simulink model "xz_packaging_automatic"  (R2025b)
settings: Solver=ode15s  StartTime=0.0  StopTime=10.45  MaxStep=0.001  RelTol=1e-6  AbsTol=1e-9
model workspace: external: MATLAB File xz_packaging_automatic_DataFile.m (data not in the file)
values from neighbouring files (symbols this model uses):
  payloadMass_kg = 0.25    [xz_packaging_automatic_DataFile.m]
undefined symbols (not defined in the file or in its folder): smiData, X, Y, Z
libraries: sm_lib x2549, nesl_utility x31
(part 1 of 38)
settings Model: Creator=Asus  LastModifiedBy=Asus

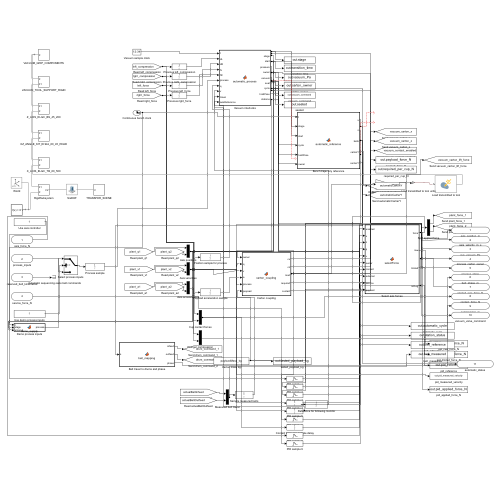
[thumbnail: Simulink's stored preview of the top-level diagram]
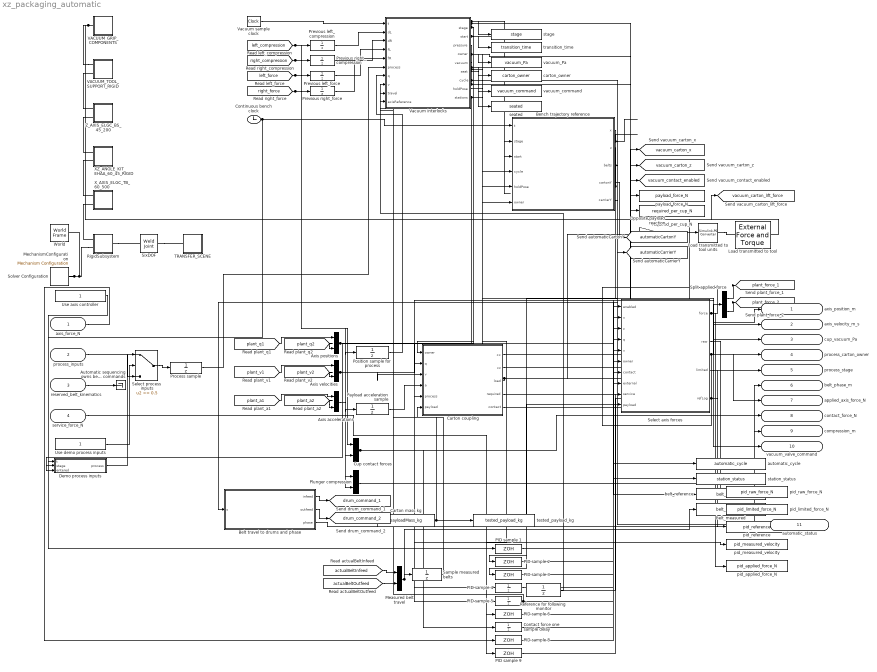
== system xz_packaging_automatic ==
  axis_force_N : Inport  PortDimensions=2
  process_inputs : Inport  Port=2  PortDimensions=12
  reserved_belt_kinematics : Inport  Port=3  PortDimensions=6
  service_force_N : Inport  Port=4  PortDimensions=2
  Automatic sequencing owns belt commands : Terminator
  Axis accelerations : Mux  Inputs=2
  Axis positions : Mux  Inputs=2
  Axis velocities : Mux  Inputs=2
  Belt travel to drums and phase : MATLAB Function  TreatAsAtomicUnit=on
  Bench trajectory reference : MATLAB Function  TreatAsAtomicUnit=on
  Carton coupling : MATLAB Function  TreatAsAtomicUnit=on
  Carton mass kg : Constant  Value=payloadMass_kg
  Contact force one sample delay : UnitDelay  SampleTime=0.001  HasFrameUpgradeWarning=on
  Continuous bench clock : Clock
  Cup contact forces : Mux  Inputs=2
  Demo process inputs : MATLAB Function  TreatAsAtomicUnit=on
  Load transmitted to tool : sm_lib/Forces and Torques/External Force and Torque  EnableForceX=off  EnableForceY=off  EnableForceZ=off  EnableForce=on  ForceResolutionFrame=World  EnableTorqueX=off  EnableTorqueY=off  EnableTorqueZ=off  EnableTorque=off  TorqueResolutionFrame=AttachedFrame
  Load transmitted to tool units : nesl_utility/Simulink-PS Converter  PhysicalDomain=network_engine_domain  SubClassName=ps_input  LeftPortType=input  RightPortType=output  PseudoPeriodic=off  Frequencies=[]  NoiseDistribution=none  NoiseParameters=[]  Unit=N  AffineConversion=off  FilteringAndDerivatives=provide  SimscapeFilterOrder=1  InputFilterTimeConstant=0.001  UdotUserProvided=0
  Measured belt travel : Mux  Inputs=2
  MechanismConfiguration : sm_lib/Utilities/Mechanism Configuration  UniformGravity=Constant  GravityVector=[0 0 -9.8066499999999994]  GravityVectorUnits=m/s^2  LinearizationDelta=0.001  JointModeTransitionNonlinearIterations=2
  Opposite payload reaction : Gain  Gain=-1
  PID sample {1..3,6,8..9} (6 alike) : ZeroOrderHold  SampleTime=0.001
  PID sample 4 : UnitDelay  InitialCondition=[0.05;0.024]  SampleTime=0.001  HasFrameUpgradeWarning=on
  PID sample 5 : UnitDelay  SampleTime=0.001  HasFrameUpgradeWarning=on
  Payload acceleration sample : UnitDelay  SampleTime=0.001  HasFrameUpgradeWarning=on
  Plunger compression : Mux  Inputs=2
  Position sample for process : UnitDelay  SampleTime=0.001  HasFrameUpgradeWarning=on
  Previous left_compression : UnitDelay  SampleTime=0.001  HasFrameUpgradeWarning=on
  Previous left_force : UnitDelay  SampleTime=0.001  HasFrameUpgradeWarning=on
  Previous right_compression : UnitDelay  SampleTime=0.001  HasFrameUpgradeWarning=on
  Previous right_force : UnitDelay  SampleTime=0.001  HasFrameUpgradeWarning=on
  Process sample : UnitDelay  SampleTime=0.001  HasFrameUpgradeWarning=on
  Reference for following monitor : UnitDelay  InitialCondition=[0.05 0 0;0.024 0 0]  SampleTime=0.001  HasFrameUpgradeWarning=on
  RigidSubsystem : Subsystem
  Sample measured belts : UnitDelay  SampleTime=0.001  HasFrameUpgradeWarning=on
  Select axis forces : MATLAB Function  TreatAsAtomicUnit=on
  Select process inputs : Switch  Threshold=0.5  SaturateOnIntegerOverflow=off  InputSameDT=off
  SixDOF : sm_lib/Joints/Weld Joint  JointMode=Normal  CompositeWrenchDir=FollowerOnBase  CompositeWrenchFrame=BaseFrame  SenseConstraintForce=off  SenseConstraintTorque=off  SenseTotalForce=off  SenseTotalTorque=off
  Solver Configuration : nesl_utility/Solver Configuration  PhysicalDomain=network_engine_domain  SubClassName=solver  LeftPortType=input  RightPortType=generic  Tones=[]  Harmonics=[]  SimulateNoise=off  Profile=off  UseLocalSampling=off  EnableSwitchedLinearOptims=on  FrequencyDomain=off  UseCCode=off  RelTol=0.001  AbsTol=0.001  MinStep=1e-09  ToWorkspace=off  RevertToSquareIcSolve=off  NumHomotopyIterations=100  PhasorMode=off  PhasorModeNumHarmonics=1  ConsistencySolver=NEWTON_XTOL_AFTER_FTOL  IndexReductionMethod=DerivativeReplacement  DoDC=off  ResidualTolerance=1e-09  ConsistencyTolSource=GLOBAL  ConsistencyAbsTol=0.001  ConsistencyRelTol=0.001  ConsistencyTolFactor=0.001  UseLocalSolver=off  LocalSolverChoice=NE_BACKWARD_EULER_ADVANCER  ResolveIndetEquations=on  FunctionEvalNumThread=1  LocalSolverSampleTime=0.001  DoFixedCost=off  MaxNonlinIter=3  MaxModeIter=2  ComputeImpulses=off  ImpulseIterations=2  LinearAlgebra=auto  LinearAlgebraNumThread=0  EquationFormulation=NE_TIME_EF  DelaysMemoryBudget=1024  AutomaticFiltering=on  FilteringTimeConstant=0.001  PartitionStorageMethod=AS_NEEDED  PartitionMemoryBudget=1024  PartitionMethod=ROBUST  MultibodyUseLocalSolver=off  MultibodyLocalSolverChoice=ODE1  MultibodyLocalSolverSampleTime=0.001
  Split applied force : Demux  Outputs=2
  TRANSFER_SCENE : Subsystem
  Use axis controller : Constant
  Use demo process inputs : Constant
  VACUUM_GRIP_COMPONENTS : Subsystem
  VACUUM_TOOL_SUPPORT_RIGID : Subsystem
  Vacuum interlocks : MATLAB Function  TreatAsAtomicUnit=on
  Vacuum sample clock : DigitalClock  SampleTime=0.001
  World : sm_lib/Frames and Transforms/World Frame
  XZ_ANGLE_KIT_EHAA_60_45_RIGID : Subsystem
  X_AXIS_ELGC_TB_60_500 : Subsystem
  Z_AXIS_ELGC_BS_45_200 : Subsystem
  automatic_cycle : ToWorkspace  VariableName=automatic_cycle  SaveFormat=Timeseries  SampleTime=-1
  belt_measured : ToWorkspace  VariableName=belt_measured  SaveFormat=Timeseries  SampleTime=-1
  belt_reference : ToWorkspace  VariableName=belt_reference  SaveFormat=Timeseries  SampleTime=-1
  carton_owner : ToWorkspace  VariableName=carton_owner  SaveFormat=Timeseries  SampleTime=-1
  payload_force_N : ToWorkspace  VariableName=payload_force_N  SaveFormat=Timeseries  SampleTime=-1
  pid_applied_force_N : ToWorkspace  VariableName=pid_applied_force_N  SaveFormat=Timeseries  SampleTime=-1
  pid_limited_force_N : ToWorkspace  VariableName=pid_limited_force_N  SaveFormat=Timeseries  SampleTime=-1
  pid_measured_velocity : ToWorkspace  VariableName=pid_measured_velocity  SaveFormat=Timeseries  SampleTime=-1
  pid_raw_force_N : ToWorkspace  VariableName=pid_raw_force_N  SaveFormat=Timeseries  SampleTime=-1
  pid_reference : ToWorkspace  VariableName=pid_reference  SaveFormat=Timeseries  SampleTime=-1
  required_per_cup_N : ToWorkspace  VariableName=required_per_cup_N  SaveFormat=Timeseries  SampleTime=-1
  seated : ToWorkspace  VariableName=seated  SaveFormat=Timeseries  SampleTime=-1
  stage : ToWorkspace  VariableName=stage  SaveFormat=Timeseries  SampleTime=-1
  station_status : ToWorkspace  VariableName=station_status  SaveFormat=Timeseries  SampleTime=-1
  tested_payload_kg : ToWorkspace  VariableName=tested_payload_kg  SaveFormat=Timeseries  SampleTime=-1
  transition_time : ToWorkspace  VariableName=transition_time  SaveFormat=Timeseries  SampleTime=-1
  vacuum_Pa : ToWorkspace  VariableName=vacuum_Pa  SaveFormat=Timeseries  SampleTime=-1
  vacuum_command : ToWorkspace  VariableName=vacuum_command  SaveFormat=Timeseries  SampleTime=-1
  axis_position_m : Outport
  axis_velocity_m_s : Outport  Port=2
  cup_vacuum_Pa : Outport  Port=3
  process_carton_owner : Outport  Port=4
  process_stage : Outport  Port=5
  belt_phase_m : Outport  Port=6
  applied_axis_force_N : Outport  Port=7
  contact_force_N : Outport  Port=8
  compression_m : Outport  Port=9
  vacuum_valve_command : Outport  Port=10
  automatic_status : Outport  Port=11
  tag scope: automaticCarrierY=global, automaticCartonY=global, drum_command_1=global, drum_command_2=global, plant_force_1=global, plant_force_2=global, vacuum_carton_lift_force=global, vacuum_carton_x=global, vacuum_carton_z=global, vacuum_contact_enabled=global
  wires:
  Vacuum sample clock/1 -> Vacuum interlocks/1(t)
  Continuous bench clock/1 -> Bench trajectory reference/1(t), Demo process inputs/1(t)
  Vacuum interlocks/1(stage) -> Bench trajectory reference/2(stage), stage/1, process_stage/1, Demo process inputs/2(stage)
  Vacuum interlocks/2(start) -> Bench trajectory reference/3(start), transition_time/1, Demo process inputs/3(entered)
  Vacuum interlocks/4(owner) -> carton_owner/1, Carton coupling/1(owner), process_carton_owner/1, PID sample 6/1, Bench trajectory reference/6(owner)
  [left_compression] -> Previous left_compression/1, Plunger compression/1
  Previous left_compression/1 -> Vacuum interlocks/2(dL)
  [right_compression] -> Previous right_compression/1, Plunger compression/2
  Previous right_compression/1 -> Vacuum interlocks/3(dR)
  [left_force] -> Previous left_force/1, Cup contact forces/1
  Previous left_force/1 -> Vacuum interlocks/4(fL)
  [right_force] -> Previous right_force/1, Cup contact forces/2
  Previous right_force/1 -> Vacuum interlocks/5(fR)
  Bench trajectory reference/1(x) -> PID sample 2/1
  Bench trajectory reference/2(z) -> PID sample 3/1
  Opposite payload reaction/1 -> Load transmitted to tool units/1
  Vacuum interlocks/3(pressure) -> vacuum_Pa/1, cup_vacuum_Pa/1
  Vacuum interlocks/5(vacuum) -> vacuum_command/1, vacuum_valve_command/1
  Vacuum interlocks/6(seat) -> seated/1
  Use demo process inputs/1 -> Select process inputs/2
  process_inputs/1 -> Select process inputs/3
  [plant_q1] -> Axis positions/1
  [plant_q2] -> Axis positions/2
  [plant_v1] -> Axis velocities/1
  [plant_v2] -> Axis velocities/2
  [plant_a1] -> Axis accelerations/1
  [plant_a2] -> Axis accelerations/2
  Axis accelerations/1 -> Payload acceleration sample/1
  Axis positions/1 -> Position sample for process/1, Carton coupling/2(q), axis_position_m/1, PID sample 4/1
  Select process inputs/1 -> Process sample/1
  Process sample/1 -> Vacuum interlocks/6(process)
  Position sample for process/1 -> Vacuum interlocks/7(q)
  Axis velocities/1 -> Carton coupling/3(v), axis_velocity_m_s/1, PID sample 5/1, pid_measured_velocity/1
  Payload acceleration sample/1 -> Carton coupling/4(a)
  Carton coupling/1(cx) -> [vacuum_carton_x]
  Carton coupling/2(cz) -> [vacuum_carton_z]
  Carton coupling/3(load) -> [vacuum_carton_lift_force], Opposite payload reaction/1, payload_force_N/1
  Carton coupling/4(required) -> required_per_cup_N/1
  Carton coupling/5(contact) -> [vacuum_contact_enabled]
  Cup contact forces/1 -> contact_force_N/1, Contact force one sample delay/1
  Select axis forces/1(force) -> Split applied force/1, applied_axis_force_N/1, pid_applied_force_N/1
  Split applied force/1 -> [plant_force_1]
  Split applied force/2 -> [plant_force_2]
  Belt travel to drums and phase/1(infeed) -> [drum_command_1]
  Belt travel to drums and phase/2(outfeed) -> [drum_command_2]
  Belt travel to drums and phase/3(phase) -> belt_phase_m/1
  Plunger compression/1 -> compression_m/1
  Use axis controller/1 -> PID sample 1/1
  PID sample 1/1 -> Select axis forces/1(enabled)
  PID sample 2/1 -> Select axis forces/2(x)
  PID sample 3/1 -> Select axis forces/3(z)
  PID sample 4/1 -> Select axis forces/4(q)
  PID sample 5/1 -> Select axis forces/5(v), Vacuum interlocks/8(v)
  PID sample 6/1 -> Select axis forces/6(owner)
  Contact force one sample delay/1 -> Select axis forces/7(contact)
  axis_force_N/1 -> PID sample 8/1
  PID sample 8/1 -> Select axis forces/8(external)
  service_force_N/1 -> PID sample 9/1
  PID sample 9/1 -> Select axis forces/9(service)
  Select axis forces/2(raw) -> pid_raw_force_N/1
  Select axis forces/3(limited) -> pid_limited_force_N/1
  Select axis forces/4(refLog) -> pid_reference/1, Reference for following monitor/1
  Carton mass kg/1 -> Carton coupling/6(payload), Select axis forces/10(payload), tested_payload_kg/1
  Demo process inputs/1(process) -> Select process inputs/1
  Vacuum interlocks/7(cycle) -> Bench trajectory reference/4(cycle), automatic_cycle/1, automatic_status/1
  Vacuum interlocks/8(holdPose) -> Bench trajectory reference/5(holdPose)
  Vacuum interlocks/9(stations) -> Carton coupling/5(process), station_status/1
  Bench trajectory reference/3(belts) -> Belt travel to drums and phase/1(s), belt_reference/1
  reserved_belt_kinematics/1 -> Automatic sequencing owns belt commands/1
  [actualBeltInfeed] -> Measured belt travel/1
  [actualBeltOutfeed] -> Measured belt travel/2
  Measured belt travel/1 -> Sample measured belts/1, belt_measured/1
  Sample measured belts/1 -> Vacuum interlocks/9(travel)
  Bench trajectory reference/4(cartonY) -> [automaticCartonY]
  Bench trajectory reference/5(carrierY) -> [automaticCarrierY]
  Reference for following monitor/1 -> Vacuum interlocks/10(axisReference)
  connections:
  RigidSubsystem/LConn2 -- MechanismConfiguration/RConn1 -- Solver Configuration/RConn1 -- World/RConn1
  RigidSubsystem/LConn1 -- X_AXIS_ELGC_TB_60_500/LConn2
  SixDOF/RConn1 -- TRANSFER_SCENE/LConn1
  XZ_ANGLE_KIT_EHAA_60_45_RIGID/LConn2 -- X_AXIS_ELGC_TB_60_500/LConn1
  XZ_ANGLE_KIT_EHAA_60_45_RIGID/LConn1 -- Z_AXIS_ELGC_BS_45_200/LConn2
  VACUUM_TOOL_SUPPORT_RIGID/LConn1 -- VACUUM_GRIP_COMPONENTS/LConn1 -- Load transmitted to tool/RConn1
  VACUUM_TOOL_SUPPORT_RIGID/LConn2 -- Z_AXIS_ELGC_BS_45_200/LConn1
  RigidSubsystem/RConn1 -- SixDOF/LConn1
  Load transmitted to tool units/RConn1 -- Load transmitted to tool/LConn1

== system xz_packaging_automatic/RigidSubsystem ==
  BOLTED_FRAME_STRUCTURE_RIGID : Subsystem
  MACHINE_LAYOUT_RIGID : Subsystem
  SV_FLEX_Q000_RIGID : Subsystem
  SV_STATIONARY_RIGID : Subsystem
  Transform : sm_lib/Frames and Transforms/Rigid Transform  RotationMethod=ArbitraryAxis  FollAlignAxisA=+X  BaseAlignAxisA=+Y  FollAlignAxisB=+Y  BaseAlignAxisB=+Z  RotationStandardAxis=+Z  RotationAngle=smiData.RigidTransform(26).angle  RotationAngleUnits=rad  RotationArbitraryAxis=smiData.RigidTransform(26).axis  RotationSequenceAxes=FollowerAxes  RotationSequence=XYX  RotationSequenceAngles=[0 0 0]  RotationSequenceAnglesUnits=deg  RotationMatrix=[1 0 0;0 1 0;0 0 1]  Quaternion=[1 0 0 0]  TranslationMethod=Cartesian  TranslationCartesianOffset=smiData.RigidTransform(26).translation  TranslationCartesianOffsetUnits=mm  TranslationStandardAxis=+Z  TranslationStandardOffset=0  TranslationStandardOffsetUnits=m  TranslationROffset=0  TranslationROffsetUnits=m  TranslationThetaOffset=0  TranslationThetaOffsetUnits=deg  TranslationZOffset=0  TranslationZOffsetUnits=m
  Transform1 : sm_lib/Frames and Transforms/Rigid Transform  RotationMethod=ArbitraryAxis  FollAlignAxisA=+X  BaseAlignAxisA=+Y  FollAlignAxisB=+Y  BaseAlignAxisB=+Z  RotationStandardAxis=+Z  RotationAngle=smiData.RigidTransform(843).angle  RotationAngleUnits=rad  RotationArbitraryAxis=smiData.RigidTransform(843).axis  RotationSequenceAxes=FollowerAxes  RotationSequence=XYX  RotationSequenceAngles=[0 0 0]  RotationSequenceAnglesUnits=deg  RotationMatrix=[1 0 0;0 1 0;0 0 1]  Quaternion=[1 0 0 0]  TranslationMethod=Cartesian  TranslationCartesianOffset=smiData.RigidTransform(843).translation  TranslationCartesianOffsetUnits=mm  TranslationStandardAxis=+Z  TranslationStandardOffset=0  TranslationStandardOffsetUnits=m  TranslationROffset=0  TranslationROffsetUnits=m  TranslationThetaOffset=0  TranslationThetaOffsetUnits=deg  TranslationZOffset=0  TranslationZOffsetUnits=m
  Transform2 : sm_lib/Frames and Transforms/Rigid Transform  RotationMethod=ArbitraryAxis  FollAlignAxisA=+X  BaseAlignAxisA=+Y  FollAlignAxisB=+Y  BaseAlignAxisB=+Z  RotationStandardAxis=+Z  RotationAngle=smiData.RigidTransform(857).angle  RotationAngleUnits=rad  RotationArbitraryAxis=smiData.RigidTransform(857).axis  RotationSequenceAxes=FollowerAxes  RotationSequence=XYX  RotationSequenceAngles=[0 0 0]  RotationSequenceAnglesUnits=deg  RotationMatrix=[1 0 0;0 1 0;0 0 1]  Quaternion=[1 0 0 0]  TranslationMethod=Cartesian  TranslationCartesianOffset=smiData.RigidTransform(857).translation  TranslationCartesianOffsetUnits=mm  TranslationStandardAxis=+Z  TranslationStandardOffset=0  TranslationStandardOffsetUnits=m  TranslationROffset=0  TranslationROffsetUnits=m  TranslationThetaOffset=0  TranslationThetaOffsetUnits=deg  TranslationZOffset=0  TranslationZOffsetUnits=m
  Transform3 : sm_lib/Frames and Transforms/Rigid Transform  RotationMethod=ArbitraryAxis  FollAlignAxisA=+X  BaseAlignAxisA=+Y  FollAlignAxisB=+Y  BaseAlignAxisB=+Z  RotationStandardAxis=+Z  RotationAngle=smiData.RigidTransform(858).angle  RotationAngleUnits=rad  RotationArbitraryAxis=smiData.RigidTransform(858).axis  RotationSequenceAxes=FollowerAxes  RotationSequence=XYX  RotationSequenceAngles=[0 0 0]  RotationSequenceAnglesUnits=deg  RotationMatrix=[1 0 0;0 1 0;0 0 1]  Quaternion=[1 0 0 0]  TranslationMethod=Cartesian  TranslationCartesianOffset=smiData.RigidTransform(858).translation  TranslationCartesianOffsetUnits=mm  TranslationStandardAxis=+Z  TranslationStandardOffset=0  TranslationStandardOffsetUnits=m  TranslationROffset=0  TranslationROffsetUnits=m  TranslationThetaOffset=0  TranslationThetaOffsetUnits=deg  TranslationZOffset=0  TranslationZOffsetUnits=m
  Transform4 : sm_lib/Frames and Transforms/Rigid Transform  RotationMethod=ArbitraryAxis  FollAlignAxisA=+X  BaseAlignAxisA=+Y  FollAlignAxisB=+Y  BaseAlignAxisB=+Z  RotationStandardAxis=+Z  RotationAngle=smiData.RigidTransform(859).angle  RotationAngleUnits=rad  RotationArbitraryAxis=smiData.RigidTransform(859).axis  RotationSequenceAxes=FollowerAxes  RotationSequence=XYX  RotationSequenceAngles=[0 0 0]  RotationSequenceAnglesUnits=deg  RotationMatrix=[1 0 0;0 1 0;0 0 1]  Quaternion=[1 0 0 0]  TranslationMethod=Cartesian  TranslationCartesianOffset=smiData.RigidTransform(859).translation  TranslationCartesianOffsetUnits=mm  TranslationStandardAxis=+Z  TranslationStandardOffset=0  TranslationStandardOffsetUnits=m  TranslationROffset=0  TranslationROffsetUnits=m  TranslationThetaOffset=0  TranslationThetaOffsetUnits=deg  TranslationZOffset=0  TranslationZOffsetUnits=m
  Transform5 : sm_lib/Frames and Transforms/Rigid Transform  RotationMethod=ArbitraryAxis  FollAlignAxisA=+X  BaseAlignAxisA=+Y  FollAlignAxisB=+Y  BaseAlignAxisB=+Z  RotationStandardAxis=+Z  RotationAngle=smiData.RigidTransform(860).angle  RotationAngleUnits=rad  RotationArbitraryAxis=smiData.RigidTransform(860).axis  RotationSequenceAxes=FollowerAxes  RotationSequence=XYX  RotationSequenceAngles=[0 0 0]  RotationSequenceAnglesUnits=deg  RotationMatrix=[1 0 0;0 1 0;0 0 1]  Quaternion=[1 0 0 0]  TranslationMethod=Cartesian  TranslationCartesianOffset=smiData.RigidTransform(860).translation  TranslationCartesianOffsetUnits=mm  TranslationStandardAxis=+Z  TranslationStandardOffset=0  TranslationStandardOffsetUnits=m  TranslationROffset=0  TranslationROffsetUnits=m  TranslationThetaOffset=0  TranslationThetaOffsetUnits=deg  TranslationZOffset=0  TranslationZOffsetUnits=m
  Transform6 : sm_lib/Frames and Transforms/Rigid Transform  RotationMethod=ArbitraryAxis  FollAlignAxisA=+X  BaseAlignAxisA=+Y  FollAlignAxisB=+Y  BaseAlignAxisB=+Z  RotationStandardAxis=+Z  RotationAngle=smiData.RigidTransform(861).angle  RotationAngleUnits=rad  RotationArbitraryAxis=smiData.RigidTransform(861).axis  RotationSequenceAxes=FollowerAxes  RotationSequence=XYX  RotationSequenceAngles=[0 0 0]  RotationSequenceAnglesUnits=deg  RotationMatrix=[1 0 0;0 1 0;0 0 1]  Quaternion=[1 0 0 0]  TranslationMethod=Cartesian  TranslationCartesianOffset=smiData.RigidTransform(861).translation  TranslationCartesianOffsetUnits=mm  TranslationStandardAxis=+Z  TranslationStandardOffset=0  TranslationStandardOffsetUnits=m  TranslationROffset=0  TranslationROffsetUnits=m  TranslationThetaOffset=0  TranslationThetaOffsetUnits=deg  TranslationZOffset=0  TranslationZOffsetUnits=m
  Transform7 : sm_lib/Frames and Transforms/Rigid Transform  RotationMethod=ArbitraryAxis  FollAlignAxisA=+X  BaseAlignAxisA=+Y  FollAlignAxisB=+Y  BaseAlignAxisB=+Z  RotationStandardAxis=+Z  RotationAngle=smiData.RigidTransform(862).angle  RotationAngleUnits=rad  RotationArbitraryAxis=smiData.RigidTransform(862).axis  RotationSequenceAxes=FollowerAxes  RotationSequence=XYX  RotationSequenceAngles=[0 0 0]  RotationSequenceAnglesUnits=deg  RotationMatrix=[1 0 0;0 1 0;0 0 1]  Quaternion=[1 0 0 0]  TranslationMethod=Cartesian  TranslationCartesianOffset=smiData.RigidTransform(862).translation  TranslationCartesianOffsetUnits=mm  TranslationStandardAxis=+Z  TranslationStandardOffset=0  TranslationStandardOffsetUnits=m  TranslationROffset=0  TranslationROffsetUnits=m  TranslationThetaOffset=0  TranslationThetaOffsetUnits=deg  TranslationZOffset=0  TranslationZOffsetUnits=m
  Transform8 : sm_lib/Frames and Transforms/Rigid Transform  RotationMethod=ArbitraryAxis  FollAlignAxisA=+X  BaseAlignAxisA=+Y  FollAlignAxisB=+Y  BaseAlignAxisB=+Z  RotationStandardAxis=+Z  RotationAngle=smiData.RigidTransform(863).angle  RotationAngleUnits=rad  RotationArbitraryAxis=smiData.RigidTransform(863).axis  RotationSequenceAxes=FollowerAxes  RotationSequence=XYX  RotationSequenceAngles=[0 0 0]  RotationSequenceAnglesUnits=deg  RotationMatrix=[1 0 0;0 1 0;0 0 1]  Quaternion=[1 0 0 0]  TranslationMethod=Cartesian  TranslationCartesianOffset=smiData.RigidTransform(863).translation  TranslationCartesianOffsetUnits=mm  TranslationStandardAxis=+Z  TranslationStandardOffset=0  TranslationStandardOffsetUnits=m  TranslationROffset=0  TranslationROffsetUnits=m  TranslationThetaOffset=0  TranslationThetaOffsetUnits=deg  TranslationZOffset=0  TranslationZOffsetUnits=m
  Transform9 : sm_lib/Frames and Transforms/Rigid Transform  RotationMethod=ArbitraryAxis  FollAlignAxisA=+X  BaseAlignAxisA=+Y  FollAlignAxisB=+Y  BaseAlignAxisB=+Z  RotationStandardAxis=+Z  RotationAngle=smiData.RigidTransform(875).angle  RotationAngleUnits=rad  RotationArbitraryAxis=smiData.RigidTransform(875).axis  RotationSequenceAxes=FollowerAxes  RotationSequence=XYX  RotationSequenceAngles=[0 0 0]  RotationSequenceAnglesUnits=deg  RotationMatrix=[1 0 0;0 1 0;0 0 1]  Quaternion=[1 0 0 0]  TranslationMethod=Cartesian  TranslationCartesianOffset=smiData.RigidTransform(875).translation  TranslationCartesianOffsetUnits=mm  TranslationStandardAxis=+Z  TranslationStandardOffset=0  TranslationStandardOffsetUnits=m  TranslationROffset=0  TranslationROffsetUnits=m  TranslationThetaOffset=0  TranslationThetaOffsetUnits=deg  TranslationZOffset=0  TranslationZOffsetUnits=m
  XZ_CARRIERS_POSE_Q000_RIGID : Subsystem
  X_AXIS_MOUNTING_SET_RIGID : Subsystem
  X_CARRIER_TRAY_MOUNT_RIGID : Subsystem
  X_FIXED_CHAIN_END_MOUNTS_RIGID : Subsystem
  F1 : PMIOPort  Side=Left
  F : PMIOPort  Port=2  Side=Left
  F2 : PMIOPort  Port=3  Side=Right
  connections:
  Transform1/LConn1 -- Transform/LConn1 -- Transform2/LConn1 -- Transform3/LConn1 -- Transform4/LConn1 -- Transform5/LConn1 -- Transform6/LConn1 -- Transform7/LConn1 -- Transform8/LConn1 -- Transform9/LConn1 -- F/RConn1
  Transform/RConn1 -- F1/RConn1
  Transform5/RConn1 -- X_FIXED_CHAIN_END_MOUNTS_RIGID/LConn1
  Transform6/RConn1 -- XZ_CARRIERS_POSE_Q000_RIGID/LConn1
  SV_STATIONARY_RIGID/LConn1 -- Transform7/RConn1
  SV_FLEX_Q000_RIGID/LConn1 -- Transform8/RConn1
  Transform9/RConn1 -- F2/RConn1
  MACHINE_LAYOUT_RIGID/LConn1 -- Transform1/RConn1
  Transform2/RConn1 -- X_AXIS_MOUNTING_SET_RIGID/LConn1
  BOLTED_FRAME_STRUCTURE_RIGID/LConn1 -- Transform3/RConn1
  Transform4/RConn1 -- X_CARRIER_TRAY_MOUNT_RIGID/LConn1

== system xz_packaging_automatic/TRANSFER_SCENE ==
  RigidSubsystem : Subsystem
  SixDOF : sm_lib/Joints/Weld Joint  JointMode=Normal  CompositeWrenchDir=FollowerOnBase  CompositeWrenchFrame=BaseFrame  SenseConstraintForce=off  SenseConstraintTorque=off  SenseTotalForce=off  SenseTotalTorque=off
  TRANSFER_SCENE_1 : Subsystem
  F : PMIOPort  Side=Left
  connections:
  SixDOF/RConn1 -- TRANSFER_SCENE_1/LConn1
  RigidSubsystem/RConn1 -- SixDOF/LConn1
  RigidSubsystem/LConn1 -- F/RConn1

== system xz_packaging_automatic/VACUUM_GRIP_COMPONENTS ==
  Prismatic : sm_lib/Joints/Prismatic Joint  JointMode=Normal  CompositeWrenchDir=FollowerOnBase  CompositeWrenchFrame=BaseFrame  SenseConstraintForce=off  SenseConstraintTorque=off  SenseTotalForce=off  SenseTotalTorque=off  PositionTargetSpecify=on  PositionTargetPriority=High  PositionTargetValue=0  PositionTargetValueUnits=m  VelocityTargetSpecify=on  VelocityTargetPriority=High  VelocityTargetValue=0  VelocityTargetValueUnits=m/s  EquilibriumPosition=-0.015972850678733032  EquilibriumPositionUnits=m  SpringStiffness=221  SpringStiffnessUnits=N/m  DampingCoefficient=3  DampingCoefficientUnits=N/(m/s)  LowerLimitSpecify=on  LowerLimitBound=0  LowerLimitBoundUnits=m  LowerLimitStiffness=5e6  LowerLimitStiffnessUnits=N/m  LowerLimitDamping=500  LowerLimitDampingUnits=N/(m/s)  LowerLimitTransitionRegionWidth=1e-7  LowerLimitTransitionRegionWidthUnits=m  UpperLimitSpecify=on  UpperLimitBound=0.002  UpperLimitBoundUnits=m  UpperLimitStiffness=5e6  UpperLimitStiffnessUnits=N/m  UpperLimitDamping=500  UpperLimitDampingUnits=N/(m/s)  UpperLimitTransitionRegionWidth=1e-7  UpperLimitTransitionRegionWidthUnits=m  TorqueActuationMode=NoTorque  MotionActuationMode=ComputedMotion  SensePosition=on  SenseVelocity=on  SenseAcceleration=off  SenseTorqueForce=off  SenseLowerLimitTorqueForce=off  SenseUpperLimitTorqueForce=off
  Prismatic1 : sm_lib/Joints/Prismatic Joint  JointMode=Normal  CompositeWrenchDir=FollowerOnBase  CompositeWrenchFrame=BaseFrame  SenseConstraintForce=off  SenseConstraintTorque=off  SenseTotalForce=off  SenseTotalTorque=off  PositionTargetSpecify=on  PositionTargetPriority=High  PositionTargetValue=0  PositionTargetValueUnits=m  VelocityTargetSpecify=on  VelocityTargetPriority=High  VelocityTargetValue=0  VelocityTargetValueUnits=m/s  EquilibriumPosition=-0.015972850678733032  EquilibriumPositionUnits=m  SpringStiffness=221  SpringStiffnessUnits=N/m  DampingCoefficient=3  DampingCoefficientUnits=N/(m/s)  LowerLimitSpecify=on  LowerLimitBound=0  LowerLimitBoundUnits=m  LowerLimitStiffness=5e6  LowerLimitStiffnessUnits=N/m  LowerLimitDamping=500  LowerLimitDampingUnits=N/(m/s)  LowerLimitTransitionRegionWidth=1e-7  LowerLimitTransitionRegionWidthUnits=m  UpperLimitSpecify=on  UpperLimitBound=0.002  UpperLimitBoundUnits=m  UpperLimitStiffness=5e6  UpperLimitStiffnessUnits=N/m  UpperLimitDamping=500  UpperLimitDampingUnits=N/(m/s)  UpperLimitTransitionRegionWidth=1e-7  UpperLimitTransitionRegionWidthUnits=m  TorqueActuationMode=NoTorque  MotionActuationMode=ComputedMotion  SensePosition=on  SenseVelocity=on  SenseAcceleration=off  SenseTorqueForce=off  SenseLowerLimitTorqueForce=off  SenseUpperLimitTorqueForce=off
  RigidSubsystem : Subsystem
  VG_LEFT_MOVING_RIGID : Subsystem
  VG_RIGHT_MOVING_RIGID : Subsystem
  left carton height offset : FromWorkspace  VariableName=benchHeightLeft  Interpolate=off  OutputAfterFinalValue=Holding final value
  left compression : nesl_utility/PS-Simulink Converter  PhysicalDomain=network_engine_domain  SubClassName=ps_output  LeftPortType=input  RightPortType=output  PseudoPeriodic=off  Frequencies=[]  VectorFormat=inherit  Unit=m  AffineConversion=off
  left compression velocity : nesl_utility/PS-Simulink Converter  PhysicalDomain=network_engine_domain  SubClassName=ps_output  LeftPortType=input  RightPortType=output  PseudoPeriodic=off  Frequencies=[]  VectorFormat=inherit  Unit=m/s  AffineConversion=off
  left normal contact : MATLAB Function  TreatAsAtomicUnit=on
  left normal force units : nesl_utility/Simulink-PS Converter  PhysicalDomain=network_engine_domain  SubClassName=ps_input  LeftPortType=input  RightPortType=output  PseudoPeriodic=off  Frequencies=[]  NoiseDistribution=none  NoiseParameters=[]  Unit=N  AffineConversion=off  FilteringAndDerivatives=provide  SimscapeFilterOrder=1  InputFilterTimeConstant=0.001  UdotUserProvided=0
  left upward contact force : sm_lib/Forces and Torques/External Force and Torque  EnableForceX=off  EnableForceY=off  EnableForceZ=on  EnableForce=off  ForceResolutionFrame=World  EnableTorqueX=off  EnableTorqueY=off  EnableTorqueZ=off  EnableTorque=off  TorqueResolutionFrame=AttachedFrame
  left_compression_m : ToWorkspace  VariableName=left_compression_m  SaveFormat=Timeseries  SampleTime=-1
  left_normal_force_N : ToWorkspace  VariableName=left_normal_force_N  SaveFormat=Timeseries  SampleTime=-1
  right carton height offset : FromWorkspace  VariableName=benchHeightRight  Interpolate=off  OutputAfterFinalValue=Holding final value
  right compression : nesl_utility/PS-Simulink Converter  PhysicalDomain=network_engine_domain  SubClassName=ps_output  LeftPortType=input  RightPortType=output  PseudoPeriodic=off  Frequencies=[]  VectorFormat=inherit  Unit=m  AffineConversion=off
  right compression velocity : nesl_utility/PS-Simulink Converter  PhysicalDomain=network_engine_domain  SubClassName=ps_output  LeftPortType=input  RightPortType=output  PseudoPeriodic=off  Frequencies=[]  VectorFormat=inherit  Unit=m/s  AffineConversion=off
  right normal contact : MATLAB Function  TreatAsAtomicUnit=on
  right normal force units : nesl_utility/Simulink-PS Converter  PhysicalDomain=network_engine_domain  SubClassName=ps_input  LeftPortType=input  RightPortType=output  PseudoPeriodic=off  Frequencies=[]  NoiseDistribution=none  NoiseParameters=[]  Unit=N  AffineConversion=off  FilteringAndDerivatives=provide  SimscapeFilterOrder=1  InputFilterTimeConstant=0.001  UdotUserProvided=0
  right upward contact force : sm_lib/Forces and Torques/External Force and Torque  EnableForceX=off  EnableForceY=off  EnableForceZ=on  EnableForce=off  ForceResolutionFrame=World  EnableTorqueX=off  EnableTorqueY=off  EnableTorqueZ=off  EnableTorque=off  TorqueResolutionFrame=AttachedFrame
  right_compression_m : ToWorkspace  VariableName=right_compression_m  SaveFormat=Timeseries  SampleTime=-1
  right_normal_force_N : ToWorkspace  VariableName=right_normal_force_N  SaveFormat=Timeseries  SampleTime=-1
  F : PMIOPort  Side=Left
  tag scope: left_compression=global, left_force=global, right_compression=global, right_force=global
  wires:
  left compression/1 -> left_compression_m/1, left normal contact/4(compression), [left_compression]
  [contact_qZ] -> left normal contact/1(qZ)
  [contact_vZ] -> left normal contact/2(vZ)
  left carton height offset/1 -> left normal contact/3(height)
  left compression velocity/1 -> left normal contact/5(speed)
  left normal contact/1(force) -> left_normal_force_N/1, left normal force units/1, [left_force]
  right compression/1 -> right_compression_m/1, right normal contact/4(compression), [right_compression]
  [contact_qZ] -> right normal contact/1(qZ)
  [contact_vZ] -> right normal contact/2(vZ)
  right carton height offset/1 -> right normal contact/3(height)
  right compression velocity/1 -> right normal contact/5(speed)
  right normal contact/1(force) -> right_normal_force_N/1, right normal force units/1, [right_force]
  [vacuum_contact_enabled] -> left normal contact/6(enabled), right normal contact/6(enabled)
  connections:
  Prismatic/LConn1 -- RigidSubsystem/RConn2
  Prismatic1/LConn1 -- RigidSubsystem/RConn1
  VG_LEFT_MOVING_RIGID/LConn1 -- Prismatic/RConn1 -- left upward contact force/RConn1
  RigidSubsystem/LConn1 -- F/RConn1
  VG_RIGHT_MOVING_RIGID/LConn1 -- Prismatic1/RConn1 -- right upward contact force/RConn1
  Prismatic/RConn2 -- left compression/LConn1
  Prismatic/RConn3 -- left compression velocity/LConn1
  left normal force units/RConn1 -- left upward contact force/LConn1
  Prismatic1/RConn2 -- right compression/LConn1
  Prismatic1/RConn3 -- right compression velocity/LConn1
  right normal force units/RConn1 -- right upward contact force/LConn1

== system xz_packaging_automatic/VACUUM_TOOL_SUPPORT_RIGID ==
  IGUS_060_50_12_MOVING_RIGID : Subsystem
  ReferenceFrame : sm_lib/Frames and Transforms/Reference Frame
  SV_TOOL_RIGID : Subsystem
  TOOL_MOUNT_FASTENERS_RIGID : Subsystem
  TOOL_SERVICE_HARDWARE_RIGID : Subsystem
  TOOL_SUPPORT_MACHINED_PARTS_RIGID : Subsystem
  Transform : sm_lib/Frames and Transforms/Rigid Transform  RotationMethod=ArbitraryAxis  FollAlignAxisA=+X  BaseAlignAxisA=+Y  FollAlignAxisB=+Y  BaseAlignAxisB=+Z  RotationStandardAxis=+Z  RotationAngle=smiData.RigidTransform(31).angle  RotationAngleUnits=rad  RotationArbitraryAxis=smiData.RigidTransform(31).axis  RotationSequenceAxes=FollowerAxes  RotationSequence=XYX  RotationSequenceAngles=[0 0 0]  RotationSequenceAnglesUnits=deg  RotationMatrix=[1 0 0;0 1 0;0 0 1]  Quaternion=[1 0 0 0]  TranslationMethod=Cartesian  TranslationCartesianOffset=smiData.RigidTransform(31).translation  TranslationCartesianOffsetUnits=mm  TranslationStandardAxis=+Z  TranslationStandardOffset=0  TranslationStandardOffsetUnits=m  TranslationROffset=0  TranslationROffsetUnits=m  TranslationThetaOffset=0  TranslationThetaOffsetUnits=deg  TranslationZOffset=0  TranslationZOffsetUnits=m
  Transform1 : sm_lib/Frames and Transforms/Rigid Transform  RotationMethod=ArbitraryAxis  FollAlignAxisA=+X  BaseAlignAxisA=+Y  FollAlignAxisB=+Y  BaseAlignAxisB=+Z  RotationStandardAxis=+Z  RotationAngle=smiData.RigidTransform(34).angle  RotationAngleUnits=rad  RotationArbitraryAxis=smiData.RigidTransform(34).axis  RotationSequenceAxes=FollowerAxes  RotationSequence=XYX  RotationSequenceAngles=[0 0 0]  RotationSequenceAnglesUnits=deg  RotationMatrix=[1 0 0;0 1 0;0 0 1]  Quaternion=[1 0 0 0]  TranslationMethod=Cartesian  TranslationCartesianOffset=smiData.RigidTransform(34).translation  TranslationCartesianOffsetUnits=mm  TranslationStandardAxis=+Z  TranslationStandardOffset=0  TranslationStandardOffsetUnits=m  TranslationROffset=0  TranslationROffsetUnits=m  TranslationThetaOffset=0  TranslationThetaOffsetUnits=deg  TranslationZOffset=0  TranslationZOffsetUnits=m
  Transform2 : sm_lib/Frames and Transforms/Rigid Transform  RotationMethod=ArbitraryAxis  FollAlignAxisA=+X  BaseAlignAxisA=+Y  FollAlignAxisB=+Y  BaseAlignAxisB=+Z  RotationStandardAxis=+Z  RotationAngle=smiData.RigidTransform(365).angle  RotationAngleUnits=rad  RotationArbitraryAxis=smiData.RigidTransform(365).axis  RotationSequenceAxes=FollowerAxes  RotationSequence=XYX  RotationSequenceAngles=[0 0 0]  RotationSequenceAnglesUnits=deg  RotationMatrix=[1 0 0;0 1 0;0 0 1]  Quaternion=[1 0 0 0]  TranslationMethod=Cartesian  TranslationCartesianOffset=smiData.RigidTransform(365).translation  TranslationCartesianOffsetUnits=mm  TranslationStandardAxis=+Z  TranslationStandardOffset=0  TranslationStandardOffsetUnits=m  TranslationROffset=0  TranslationROffsetUnits=m  TranslationThetaOffset=0  TranslationThetaOffsetUnits=deg  TranslationZOffset=0  TranslationZOffsetUnits=m
  Z_CHAIN_MOVING_END_MOUNTS_RIGID : Subsystem
  Z_GUIDE_MOVING_MOUNTS_RIGID : Subsystem
  F : PMIOPort  Side=Left
  F1 : PMIOPort  Port=2  Side=Left
  connections:
  SV_TOOL_RIGID/RConn1 -- ReferenceFrame/RConn1 -- TOOL_MOUNT_FASTENERS_RIGID/RConn1 -- TOOL_SERVICE_HARDWARE_RIGID/RConn1 -- TOOL_SUPPORT_MACHINED_PARTS_RIGID/RConn1 -- Transform/LConn1 -- Transform1/LConn1 -- Transform2/LConn1 -- Z_CHAIN_MOVING_END_MOUNTS_RIGID/RConn1 -- Z_GUIDE_MOVING_MOUNTS_RIGID/RConn1
  Transform/RConn1 -- F/RConn1
  Transform1/RConn1 -- F1/RConn1
  IGUS_060_50_12_MOVING_RIGID/LConn1 -- Transform2/RConn1
